simulink model "sensorExpoler"  (R2026a)
settings: Solver=FixedStepDiscrete  StopTime=10  FixedStep=0.001
undefined symbols (not defined in the file): Blocking, Non
libraries: amg_usbconverter_n_connect_lib x2, dspstat3 x1
settings Model: Creator=pboon  LastModifiedBy=rosva

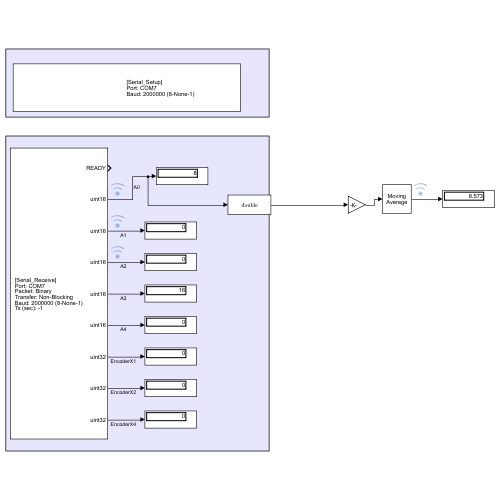
[thumbnail: Simulink's stored preview of the top-level diagram]
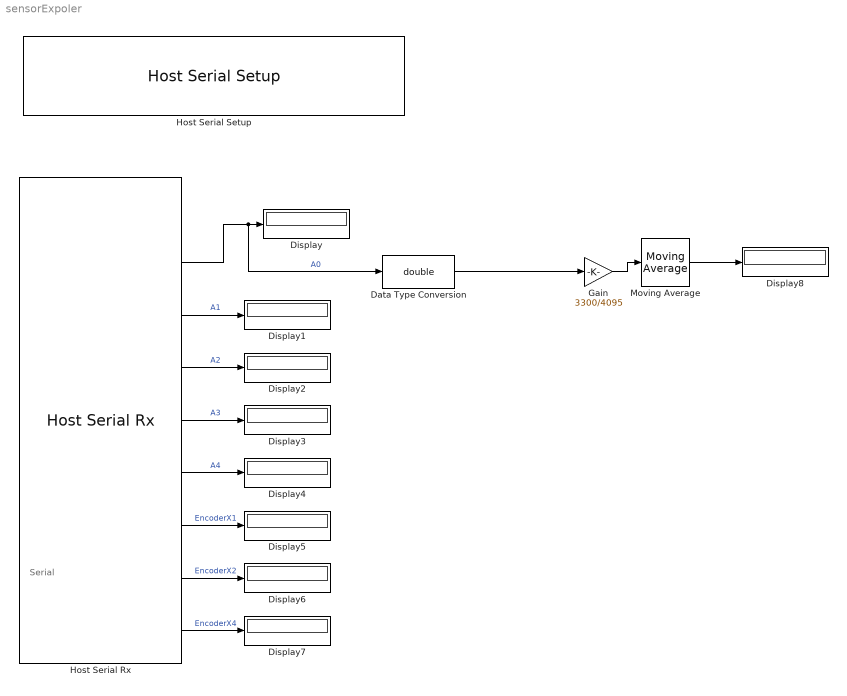
== system sensorExpoler ==
  note: Serial
  Data Type Conversion : DataTypeConversion  OutDataTypeStr=double  SaturateOnIntegerOverflow=off  RndMeth=Floor
  Display{,1..8} (9 alike) : Display
  Gain : Gain  Gain=3300/4095
  Host Serial Rx : amg_usbconverter_n_connect_lib/Host Serial Rx  conf=rx  port=<auto>  baudrate=2000000  databits=8  parity=None  stopbit=1  flowcontrol=None  transfer=Non-Blocking  timeout=5  packetmode=Binary  enableinitialvalues=off  initialvalues=[]  binheader='25'  binterminator='4E 4E'  porttype_double=0  porttype_single=0  porttype_int8=0  porttype_uint8=0  porttype_int16=0  porttype_uint16=5  porttype_int32=0  porttype_uint32=3  asciiformat='%d,%f'  rx_asciiterminator="CRLF (0x0D 0x0A - \"\\r\\n\")"  tx_asciiterminator="CRLF (0x0D 0x0A - \"\\r\\n\")"  sampletime=0.001  enablecustomportlabel=off  cinputportlabel=0  coutputportlabel=A  portpinstr=0  blockid=HostSerialRx  inputporttype=[]  inputportwidth=[]  inputportlabel={}  outputporttype=[3 5 5 5 5 5 7 7 7]  outputportwidth=[1 1 1 1 1 1 1 1 1]  outputportlabel={'READY','uint16','uint16','uint16','uint16','uint16','uint32','uint32','uint32'}  compat=0  optionstring=[]  autoport='COM7'
  Host Serial Setup : amg_usbconverter_n_connect_lib/Host Serial Setup  conf=setup  port=<auto>  baudrate=2000000  databits=8  parity=None  stopbit=1  flowcontrol=None  transfer=Blocking  timeout=2  packetmode=Binary  initialvalues=[]  binheader='7E 7E'  binterminator='03 03'  porttype_double=0  porttype_single=1  porttype_int8=0  porttype_uint8=0  porttype_int16=0  porttype_uint16=0  porttype_int32=0  porttype_uint32=2  asciiformat='%d %u %x'  rx_asciiterminator="CRLF (0x0D 0x0A - \"\\r\\n\")"  tx_asciiterminator="CRLF (0x0D 0x0A - \"\\r\\n\")"  sampletime=-1  enablecustomportlabel=off  cinputportlabel=0  coutputportlabel=A  portpinstr=0  blockid=HostSerialSetup  inputporttype=[]  inputportwidth=[]  inputportlabel={}  outputporttype=[]  outputportwidth=[]  outputportlabel={}  compat=0  optionstring=[]  autoport='COM7'
  Moving Average : dspstat3/Moving Average  Method=Sliding window  ForgettingFactorPort=off  SpecifyWindowLength=on  WindowLengthSource=Property  MaxWindowLength=20  WindowLength=500  OverlapLength=499  AllowArbitraryInputLength=off  ForgettingFactor=0.9  SimulateUsing=Interpreted execution
  wires:
  Host Serial Rx/3 -> Display1/1  "A1"
  Host Serial Rx/4 -> Display2/1  "A2"
  Host Serial Rx/5 -> Display3/1  "A3"
  Host Serial Rx/6 -> Display4/1  "A4"
  Host Serial Rx/7 -> Display5/1  "EncoderX1"
  Host Serial Rx/8 -> Display6/1  "EncoderX2"
  Host Serial Rx/9 -> Display7/1  "EncoderX4"
  Moving Average/1 -> Display8/1
  Gain/1 -> Moving Average/1
  Data Type Conversion/1 -> Gain/1
  Host Serial Rx/2 -> Data Type Conversion/1, Display/1  "A0"
